simulink model "HIamp_record_LSL_DD_vMMR"  (R2020a)
settings: Solver=VariableStepAuto  StartTime=0.0  StopTime=10000  RelTol=1e-3
libraries: LSL x1, DataAcquisition x1
settings Model: Creator=AvivaLab  LastModifiedBy=AvivaLab

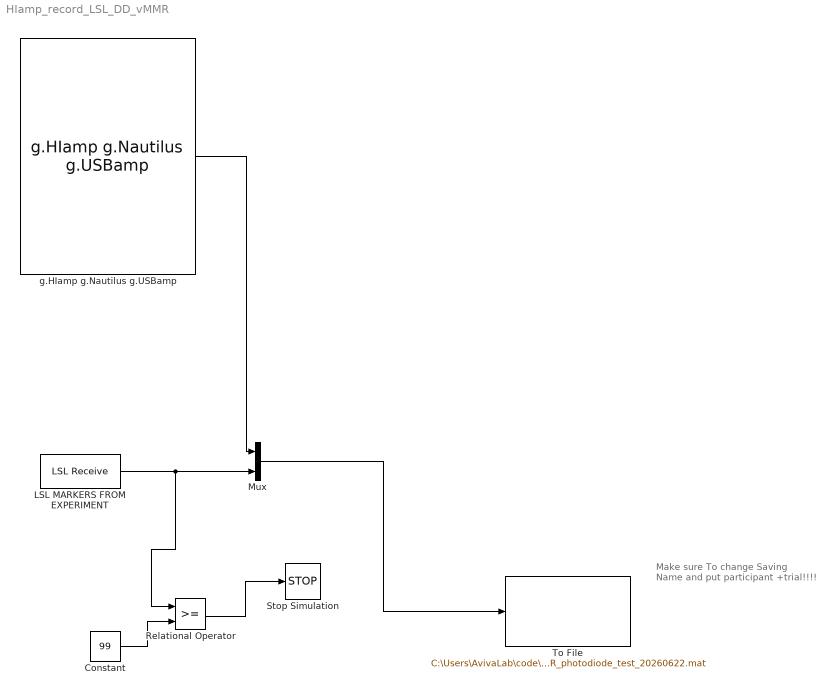
== system HIamp_record_LSL_DD_vMMR ==
  note: Make sure To change Saving Name and put participant +trial!!!!
  Constant : Constant  Value=99
  LSL MARKERS FROM EXPERIMENT : LSL/LSL Receive  noChannels=1  lslPropName=name  lslPropValue='experiment_markers'  sampleRate=1200
      settings: SourceProductName=g.HIsys
  Mux : Mux  Inputs=2
  Relational Operator : RelationalOperator  OutDataTypeStr=boolean  RndMeth=Simplest
  Stop Simulation : Stop
  To File : ToFile  Filename=C:\Users\AvivaLab\code\EEG_experiments\vMMR_EEG_PsychoPy_experiment\data\EEG_recordings\EEG_DDvMMR_photodiode_test_20260622.mat  MatrixName=EEG_data
  g.HIamp g.Nautilus g.USBamp : DataAcquisition/g.HIamp g.Nautilus g.USBamp  cfgUpdated=740155.5892  numDevices=2  deviceSR=[500 250 ]  deviceChannels=[9 4 ]  numSR=[2 ]  SRIndexPerDevice=[1 0 ]
      settings: SourceProductName=g.HIsys
  wires:
  g.HIamp g.Nautilus g.USBamp/1 -> Mux/1
  LSL MARKERS FROM EXPERIMENT/1 -> Relational Operator/1, Mux/2
  Mux/1 -> To File/1
  Relational Operator/1 -> Stop Simulation/1
  Constant/1 -> Relational Operator/2
